simulink model "case_01_fast_steady"  (R2025b)
settings: Solver=VariableStepAuto  StartTime=0.0  StopTime=30  RelTol=1e-3
settings Model: Creator=sanborkl  LastModifiedBy=sanborkl

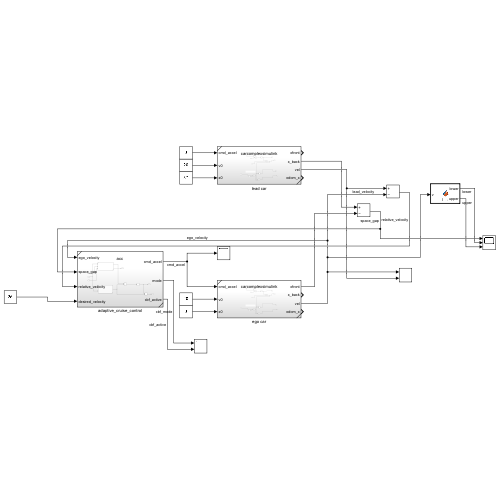
[thumbnail: Simulink's stored preview of the top-level diagram]
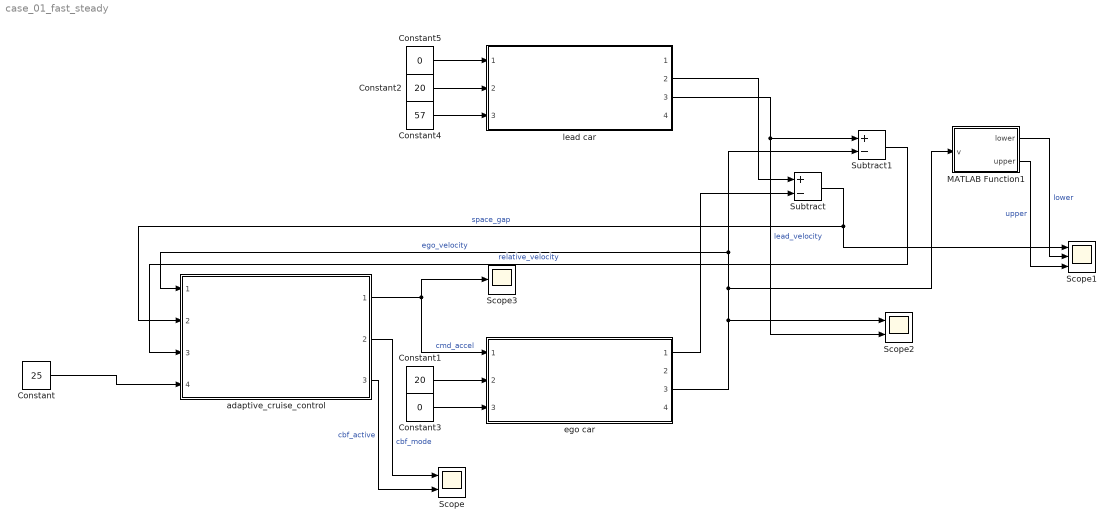
== system case_01_fast_steady ==
  Constant : Constant  Value=25
  Constant1 : Constant  Value=20
  Constant2 : Constant  Value=20
  Constant3 : Constant  Value=0
  Constant4 : Constant  Value=57
  Constant5 : Constant  Value=0
  MATLAB Function1 : MATLAB Function  TreatAsAtomicUnit=on
  Scope : Scope  NumInputPorts=2
      settings: ActiveDisplayYMinimum=0.9  ActiveDisplayYMaximum=1.1
  Scope1 : Scope  NumInputPorts=3
      settings: ActiveDisplayYMinimum=43.392637463727525  ActiveDisplayYMaximum=56.289706948474723  YLabel=m
  Scope2 : Scope  NumInputPorts=2
      settings: ActiveDisplayYMinimum=19.80824102504419  ActiveDisplayYMaximum=20.02130655277287  YLabel=m/s  DataLoggingVariableName=ScopeData2
  Scope3 : Scope
      settings: ActiveDisplayYMinimum=-0.12753716946750179  ActiveDisplayYMaximum=0.027834525207518536  YLabel=m/s^2  DataLoggingVariableName=ScopeData3
  Subtract : Sum  Inputs=+-
  Subtract1 : Sum  Inputs=+-
  adaptive_cruise_control : Subsystem  ReferencedSubsystem=acc
  ego car : Subsystem  ReferencedSubsystem=carcomplexsimulink
  lead car : Subsystem  ReferencedSubsystem=carcomplexsimulink
  wires:
  Constant5/1 -> lead car/1
  MATLAB Function1/1(lower) -> Scope1/2  "lower"
  Constant4/1 -> lead car/3
  adaptive_cruise_control/1 -> ego car/1, Scope3/1  "cmd_accel"
  Constant/1 -> adaptive_cruise_control/4
  adaptive_cruise_control/2 -> Scope/1  "cbf_mode"
  Constant3/1 -> ego car/3
  lead car/3 -> Subtract1/1, Scope2/2  "lead_velocity"
  ego car/1 -> Subtract/2
  Subtract/1 -> Scope1/1, adaptive_cruise_control/2  "space_gap"
  Constant1/1 -> ego car/2
  ego car/3 -> adaptive_cruise_control/1, Subtract1/2, MATLAB Function1/1(v), Scope2/1  "ego_velocity"
  Constant2/1 -> lead car/2
  lead car/2 -> Subtract/1
  MATLAB Function1/2(upper) -> Scope1/3  "upper"
  adaptive_cruise_control/3 -> Scope/2  "cbf_active"
  Subtract1/1 -> adaptive_cruise_control/3  "relative_velocity"

== matlab function case_01_fast_steady/MATLAB Function1 ==
  data: v input; lower output; upper output
function [lower, upper] = fcn(v)

lower = 2 * v + 5;
upper = 2 * v + 15;
